simulink model "sl_rrmc"  (Simulink 7.6)
settings: Solver=ode45  StartTime=0.0  StopTime=5.0  RelTol=1e-3
undefined symbols (not defined in the file or in its folder): DiscIntNeverNeededParam
libraries: roblocks x2
settings Model: Creator=pic  LastModifiedBy=n6334687  ExtModeAutoUpdateStatusClock=off
settings DataIOCC: LimitDataPoints=off  ReturnWorkspaceOutputs=on  SignalLoggingName=sigsOut
settings DebuggingCC: SaveWithParameterizedLinksMsg=none  SignalResolutionControl=TryResolveAllWithWarning  SolverPrmCheckMsg=none  MultiTaskDSMMsg=warning  MultiTaskCondExecSysMsg=none  StrictBusMsg=None
settings HardwareCC: TargetUnknown=on
settings RTWCC: IncludeERTFirstTime=on

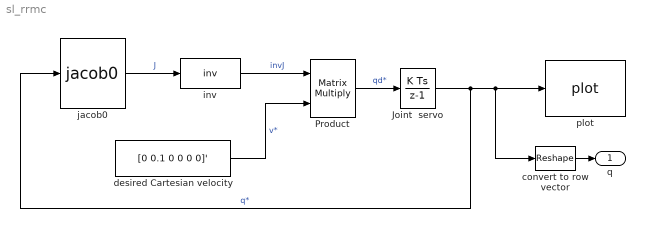
== system sl_rrmc ==
  Joint  servo : DiscreteIntegrator  InitialCondition=qn'  SampleTime=0.05  ICPrevOutput=DiscIntNeverNeededParam  ICPrevScaledInput=DiscIntNeverNeededParam
  Product : Product  Multiplication=Matrix(*)  SaturateOnIntegerOverflow=on  OutDataTypeStr=Inherit: Same as first input
  convert to row vector : Reshape  OutputDimensionality=Customize  OutputDimensions=6
  desired Cartesian velocity : Constant  Value=[0 0.1 0 0 0 0]'  VectorParams1D=off
  inv : MATLABFcn  MATLABFcn=inv  Output1D=off
  "jacob0 " : roblocks/Kinematics/jacob0   SystemSampleTime=-1  robot=p560
  plot : roblocks/Robot Graphics/plot  SystemSampleTime=-1  robot=p560
  q : Outport
  wires:
  "jacob0 "/1 -> inv/1  "J"
  Product/1 -> Joint  servo/1  "qd*"
  Joint  servo/1 -> "jacob0 "/1, plot/1, convert to row vector/1  "q*"
  inv/1 -> Product/1  "invJ"
  desired Cartesian velocity/1 -> Product/2  "v*"
  convert to row vector/1 -> q/1
